simulink model "CruiseControl_Simul"  (R2022b)
settings: Solver=FixedStepAuto  StartTime=0.0  StopTime=10  FixedStep=0.0001  RelTol=1e-3
values from neighbouring files (symbols this model uses):
  Af = 4    [CruiseControl_Initialize.m]
  Cd = 0.3    [CruiseControl_Initialize.m]
  g = 9.81    [CruiseControl_Initialize.m]
  K_I = 0.01    [CruiseControl_Initialize.m]
  K_P = 0.1    [CruiseControl_Initialize.m]
  lr = 1.8    [CruiseControl_Initialize.m]
  m = 1500    [CruiseControl_Initialize.m]
  rho = 1.225    [CruiseControl_Initialize.m]
  V_desire = 100    [CruiseControl_Initialize.m]
  xdot_0 = 60    [CruiseControl_Initialize.m]
libraries: autolibshared x1
settings Model: Creator=lego0  LastModifiedBy=lego0

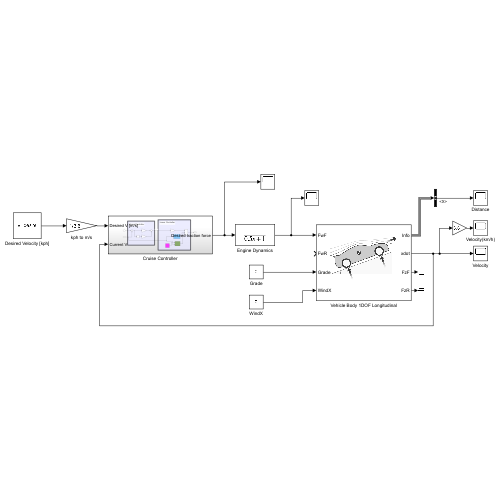
[thumbnail: Simulink's stored preview of the top-level diagram]
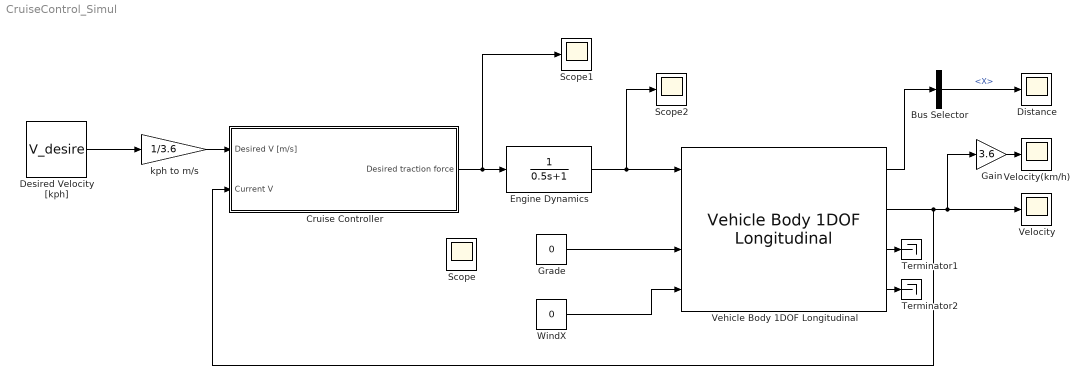
== system CruiseControl_Simul ==
  Bus Selector : BusSelector  OutputSignals=InertFrm.Cg.Disp.X
  Cruise Controller : Subsystem
  Desired Velocity [kph] : Constant  Value=V_desire
  Distance : Scope
  Engine Dynamics : TransferFcn  Denominator=[0.5 1]
  Gain : Gain  Gain=3.6
  Grade : Constant  Value=0
  Scope1 : Scope
  Scope2 : Scope
  Terminator1 : Terminator
  Terminator2 : Terminator
  Vehicle Body 1DOF Longitudinal : autolibshared/Vehicle Body 1DOF Longitudinal  VariantControl=SL  extFMode=off  extMMode=off  extTamb=off  wind3D=off  aMode=2  NF=2  NR=2  m=m  a=lf  b=lr  h=.35  Cd=Cd  Cl=0  Cpm=0  Af=Af  x_o=x_0  xdot_o=xdot_0/3.6  Pabs=101325  T=273  g=9.81
      settings: LibrarySourceBlock=vehdynlibeom/Vehicle Body 1DOF Longitudinal
  Velocity : Scope
  Velocity(km/h) : Scope
  WindX : Constant  Value=0
  kph to m/s : Gain  Gain=1/3.6
  Scope : Scope
  wires:
  Gain/1 -> Velocity(km/h)/1
  Cruise Controller/1(Desired traction force) -> Scope1/1, Engine Dynamics/1
  Desired Velocity [kph]/1 -> kph to m/s/1
  kph to m/s/1 -> Cruise Controller/1(Desired V [m/s])
  Engine Dynamics/1 -> Scope2/1, Vehicle Body 1DOF Longitudinal/1
  Grade/1 -> Vehicle Body 1DOF Longitudinal/3
  WindX/1 -> Vehicle Body 1DOF Longitudinal/4
  Vehicle Body 1DOF Longitudinal/1 -> Bus Selector/1
  Vehicle Body 1DOF Longitudinal/2 -> Cruise Controller/2(Current V), Gain/1, Velocity/1
  Vehicle Body 1DOF Longitudinal/3 -> Terminator1/1
  Vehicle Body 1DOF Longitudinal/4 -> Terminator2/1
  Bus Selector/1 -> Distance/1  "<X>"

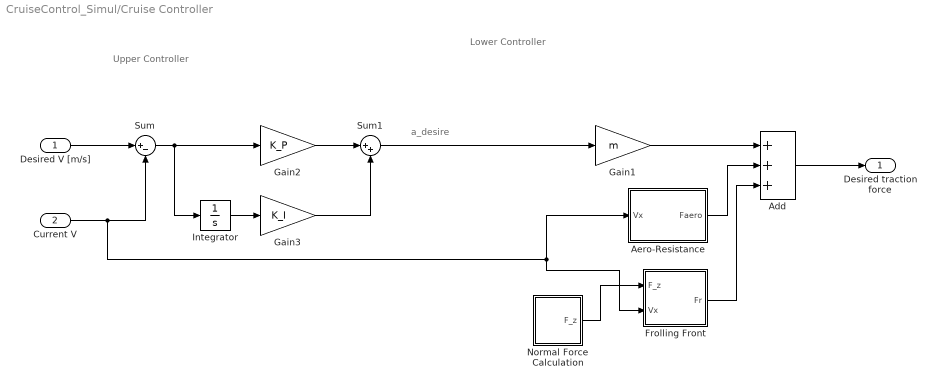
== system CruiseControl_Simul/Cruise Controller ==
  note: a_desire
  note: Upper Controller
  note: Lower Controller
  Desired V [m/s] : Inport
  Current V : Inport  Port=2
  Add : Sum  Inputs=+++
  Aero-Resistance : Subsystem
  Frolling Front : Subsystem
  Gain1 : Gain  Gain=m
  Gain2 : Gain  Gain=K_P
  Gain3 : Gain  Gain=K_I
  Integrator : Integrator
  Normal Force Calculation : Subsystem
  Sum : Sum  Inputs=|+-
  Sum1 : Sum  Inputs=|++
  Desired traction force : Outport
  wires:
  Gain2/1 -> Sum1/1
  Current V/1 -> Frolling Front/2(Vx), Aero-Resistance/1(Vx), Sum/2
  Gain3/1 -> Sum1/2
  Sum/1 -> Integrator/1, Gain2/1
  Integrator/1 -> Gain3/1
  Desired V [m/s]/1 -> Sum/1
  Sum1/1 -> Gain1/1
  Gain1/1 -> Add/1
  Add/1 -> Desired traction force/1
  Normal Force Calculation/1(F_z) -> Frolling Front/1(F_z)
  Aero-Resistance/1(Faero) -> Add/2
  Frolling Front/1(Fr) -> Add/3

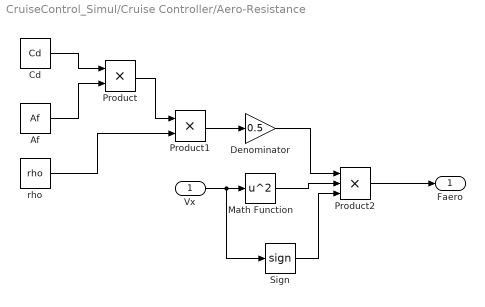
== system CruiseControl_Simul/Cruise Controller/Aero-Resistance ==
  Vx : Inport
  Af : Constant  Value=Af
  Cd : Constant  Value=Cd
  Denominator : Gain  Gain=0.5
  Math Function : Math  Operator=square  SignedPower=on
  Product : Product
  Product1 : Product
  Product2 : Product  Inputs=3
  Sign : Signum
  rho : Constant  Value=rho
  Faero : Outport  VectorParamsAs1DForOutWhenUnconnected=off
  wires:
  Af/1 -> Product/2
  Product1/1 -> Denominator/1
  Denominator/1 -> Product2/1
  Vx/1 -> Sign/1, Math Function/1
  rho/1 -> Product1/2
  Cd/1 -> Product/1
  Math Function/1 -> Product2/2
  Product/1 -> Product1/1
  Sign/1 -> Product2/3
  Product2/1 -> Faero/1

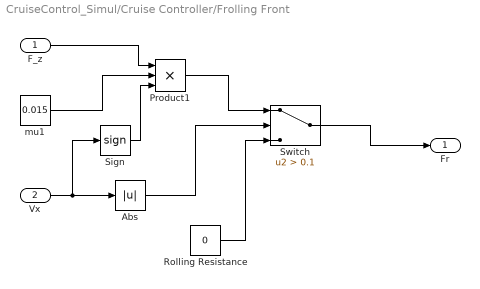
== system CruiseControl_Simul/Cruise Controller/Frolling Front ==
  F_z : Inport
  Vx : Inport  Port=2
  Abs : Abs  SaturateOnIntegerOverflow=off
  Product1 : Product  Inputs=3
  Rolling Resistance : Constant  Value=0
  Sign : Signum
  Switch : Switch  Criteria=u2 > Threshold  Threshold=0.1  SaturateOnIntegerOverflow=off  InputSameDT=off
  mu1 : Constant  Value=0.015
  Fr : Outport  VectorParamsAs1DForOutWhenUnconnected=off
  wires:
  F_z/1 -> Product1/1
  Product1/1 -> Switch/1
  Rolling Resistance/1 -> Switch/3
  mu1/1 -> Product1/2
  Vx/1 -> Sign/1, Abs/1
  Abs/1 -> Switch/2
  Sign/1 -> Product1/3
  Switch/1 -> Fr/1

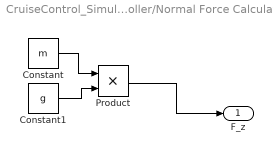
== system CruiseControl_Simul/Cruise Controller/Normal Force Calculation ==
  Constant : Constant  Value=m
  Constant1 : Constant  Value=g
  Product : Product
  F_z : Outport
  wires:
  Product/1 -> F_z/1
  Constant1/1 -> Product/2
  Constant/1 -> Product/1
